simulink model "HarnessModel_ElevationProfile"  (R2026a)
settings: Solver=daessc  StopTime=40
PreLoadFcn:
  | setupHarness_ElevationProfile
values from neighbouring files (symbols this model uses):
  s = 100    [ElevationProfile_Description.m]
undefined symbols (not defined in the file or in its folder): initial, InputLUT, RoadSurface
libraries: fl_lib x12, nesl_utility x9, sdl_lib x4
settings Model: Creator=isaacito  LastModifiedBy=isaacito
settings SimscapeCC: SimscapeLogSimulationStatistics=on  SimscapeLogLimitData=off

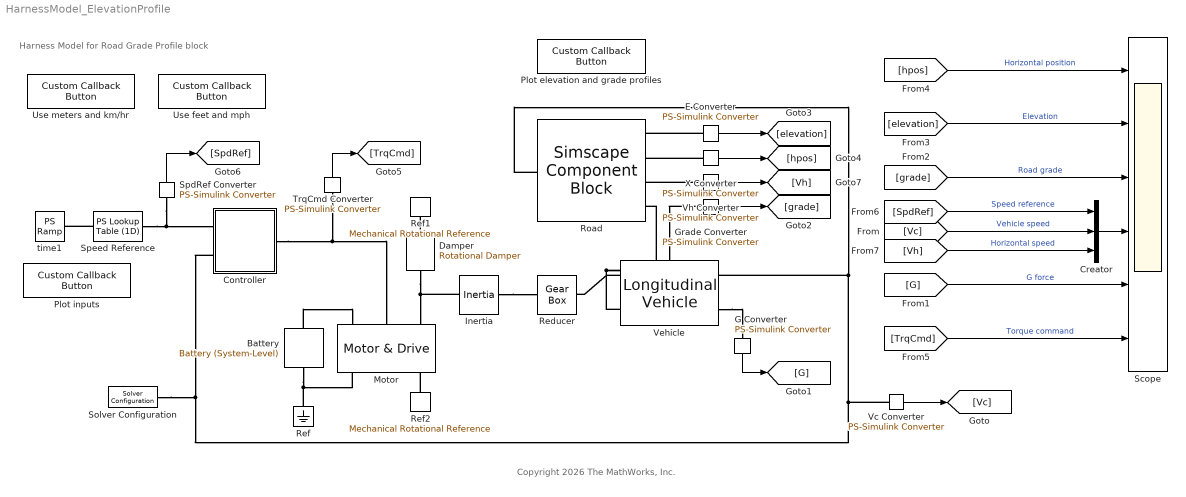
== system HarnessModel_ElevationProfile ==
  note: Harness Model for Road Grade Profile block
  note: Copyright 2026 The MathWorks, Inc.
  Battery : sdl_lib/Sources/Battery (System-Level)  Vnom=340 V  R1=0.01 Ohm  prm_AH=sdl.enum.InfiniteFinite.Infinite  AH=50 A*hr  V1=11.5 V  AH1=25 A*hr  prm_R2=sdl.enum.DisabledEnabled.Disabled  R2=2000 Ohm  thermal_port=simscape.enum.thermaleffects.omit  thermal_mass=30000 J/K  i_specify=off  i_priority=None  i=0 A  i_nominal_specify=off  i_nominal_value=1  i_nominal_unit=A  v_specify=off  v_priority=None  v=0 V  v_nominal_specify=off  v_nominal_value=1  v_nominal_unit=V  charge_specify=off  charge_priority=High  charge=50 A*hr  charge_nominal_specify=off  charge_nominal_value=1  charge_nominal_unit=A*hr  temperature_specify=off  temperature_priority=High  temperature=300 K  temperature_nominal_specify=off  temperature_nominal_value=1  temperature_nominal_unit=K
      settings: AttributesFormatString=%<Vnom> (%<Vnom_unit>)
  Controller : Subsystem
  Creator : BusCreator  Inputs=3
  Damper : sdl_lib/Couplings & Drives/Springs & Dampers/Rotational Damper  D=1e-5 N*m*s/rad  thermal_port=simscape.enum.thermaleffects.omit  thermal_mass=50 kJ/K  temperature_specify=off  temperature_priority=High  temperature=300 K  temperature_nominal_specify=off  temperature_nominal_value=1  temperature_nominal_unit=K
  E Converter : nesl_utility/PS-Simulink Converter  PhysicalDomain=network_engine_domain  SubClassName=ps_output  LeftPortType=input  RightPortType=output  PseudoPeriodic=off  Frequencies=[]  VectorFormat=inherit  Unit=ft  AffineConversion=off
  G Converter : nesl_utility/PS-Simulink Converter  PhysicalDomain=network_engine_domain  SubClassName=ps_output  LeftPortType=input  RightPortType=output  PseudoPeriodic=off  Frequencies=[]  VectorFormat=inherit  Unit=inherit  AffineConversion=off
  Grade Converter : nesl_utility/PS-Simulink Converter  PhysicalDomain=network_engine_domain  SubClassName=ps_output  LeftPortType=input  RightPortType=output  PseudoPeriodic=off  Frequencies=[]  VectorFormat=inherit  Unit=inherit  AffineConversion=off
  Inertia : fl_lib/Mechanical/Rotational Elements/Inertia  inertia=5*0.01^2 kg*m^2  num_ports=foundation.enum.numPorts2.two  w_specify=on  w_priority=None  w=0 rad/s  w_nominal_specify=off  w_nominal_value=1  w_nominal_unit=rad/s  t_specify=off  t_priority=None  t=0 N*m  t_nominal_specify=off  t_nominal_value=1  t_nominal_unit=N*m
      settings: AttributesFormatString=Priority: %<w_priority>
  Motor : sdl_lib/Engines & Motors/Motor & Drive  torque_max=160 N*m  power_max=90 kW  Tc=0.02 s  eff=100  w_eff=3750 rpm  T_eff=100 N*m  thermal_port=simscape.enum.thermaleffects.omit  thermal_mass=100 J/K  temperature_specify=off  temperature_priority=High  temperature=300 K  temperature_nominal_specify=off  temperature_nominal_value=1  temperature_nominal_unit=K
      settings: AttributesFormatString=|
      | %<torque_max> (%<torque_max_unit>)
      | %<power_max> (%<power_max_unit>)
  Plot elevation and grade profiles : CustomCallbackButton  Configuration="{\"components\":[{\"name\":\"BackgroundImageComponent\",\"settings\":{\"image\":{\"size\":[0,0],\"src\":\"default\",\"srcOrientation\":\"Right\"},\"position\":[0,0,1,1]}},{\"name\":\"ButtonStateComponent\",\"settings\":{\"buttonType\":\"momentary\",\"clickFcn\":\"plotRoadGradeProfileBlock( ...\\n  gcs + \\\"\\/Road\\\", ...\\n  UpdateModel = true, ... must update the model to get the latest values from the base workspace.\\n  InterpolationInterval = ...\\n    simscape.Value(0.2, \\\"m\\\"), ...\\n  PlotBaseData = true )\\n\",\"onValue\":1,\"position\":[0,0,1,1],\"pressDelay\":\"500\",\"pressFcn\":\"\",\"repeatInterval\":\"0\",\"states\":[{\"horizontalAlignment\":\"center\",\"image\":{\"position\":[0,0,1,1],\"size\":[1,1],\"src\":\"default\",\"srcOrientation\":\"Right\"},\"label\":{\"color\":[0.01176470588,0.01176470588,0.01176470588,1],\"icon\":{\"size\":[0,0],\"src\":\"default\",\"srcOrientation\":\"Right\"},\"iconOffset\":0,\"iconPlacement\":\"left\",\"opacity\":1,\"show\":true,\"text\":{\"content\":\"Plot profiles\",\"font\":\"Helvetica\"}},\"labelOffset\":[0,0],\"verticalAlignment\":\"middle\"},{\"horizontalAlignment\":\"center\",\"image\":{\"position\":[0,0,1,1],\"size\":[1,1],\"src\":\"default\",\"srcOrientation\":\"Right\"},\"label\":{\"color\":[0.01176470588,0.01176470588,0.01176470588,1],\"icon\":{\"size\":[0,0],\"src\":\"default\",\"srcOrientation\":\"Right\"},\"iconOffset\":0,\"iconPlacement\":\"left\",\"opacity\":1,\"show\":true,\"text\":{\"content\":\"Plot profiles\",\"font\":\"Helvetica\"}},\"labelOffset\":[0,0],\"verticalAlignment\":\"middle\"},{\"horizontalAlignment\":\"center\",\"image\":{\"position\":[0,0,1,1],\"size\":[1,1],\"src\":\"default\",\"srcOrientation\":\"Right\"},\"label\":{\"color\":[0.01176470588,0.01176470588,0.01176470588,1],\"icon\":{\"size\":[0,0],\"src\":\"default\",\"srcOrientation\":\"Right\"},\"iconOffset\":0,\"iconPlacement\":\"left\",\"opacity\":1,\"show\":true,\"text\":{\"content\":\"Plot profiles\",\"font\":\"Helvetica\"}},\"labelOffset\":[0,0],\"verticalAlignment\":\"middle\"},{\"horizontalAlignment\":\"center\",\"image\":{\"position\":[0,0,1,1],\"size\":[1,1],\"src\":\"default\",\"srcOrientation\":\"Right\"},\"label\":{\"color\":[0.01176470588,0.01176470588,0.01176470588,1],\"icon\":{\"size\":[0,0],\"src\":\"default\",\"srcOrientation\":\"Right\"},\"iconOffset\":0,\"iconPlacement\":\"left\",\"opacity\":1,\"show\":true,\"text\":{\"content\":\"Plot profiles\",\"font\":\"Helvetica\"}},\"labelOffset\":[0,0],\"verticalAlignment\":\"middle\"}]}},{\"name\":\"ForegroundImageComponent\",\"settings\":{\"image\":{\"size\":[0,0],\"src\":\"default\",\"srcOrientation\":\"Right\"},\"isForeground\":1,\"position\":[0,0,1,1]}}],\"derived\":{\"blockParameters\":{\"AutoActivate\":true,\"ButtonText\":\"Plot profiles\",\"ButtonType\":\"Momentary\",\"ClickFcn\":\"plotRoadGradeProfileBlock( ...\\n  gcs + \\\"\\/Road\\\", ...\\n  UpdateModel = true, ... must update the model to get the latest values from the base workspace.\\n  InterpolationInterval = ...\\n    simscape.Value(0.2, \\\"m\\\"), ...\\n  PlotBaseData = true )\\n\",\"OnValue\":1,\"PressDelay\":\"500\",\"PressFcn\":\"\",\"RepeatInterval\":\"0\",\"fixedAspectRatio\":\"off\"}},\"settings\":{\"BindingType\":\"standalone\",\"autoActivate\":true,\"backgroundColor\":[244,244,244,1],\"backgroundOffset\":0.2,\"backgroundOpacity\":1,\"fixedAspectRatio\":\"off\",\"foregroundColor\":[0.01176470588,0.01176470588,0.01176470588,1],\"migratedFromLegacy\":true,\"useBackgroundColor\":true,\"variant\":\"callback\",\"version\":\"R2025a\"},\"type\":\"Button\"}"  CustomBackgroundColor="{\"color\":[0.9568627451,0.9568627451,0.9568627451],\"show\":true}"
  Plot inputs : CustomCallbackButton  Configuration="{\"components\":[{\"name\":\"BackgroundImageComponent\",\"settings\":{\"image\":{\"size\":[0,0],\"src\":\"default\",\"srcOrientation\":\"Right\"},\"position\":[0,0,1,1]}},{\"name\":\"ButtonStateComponent\",\"settings\":{\"buttonType\":\"momentary\",\"clickFcn\":\"bevutil1.SignalUtil.plotLookupTable1DBlocks(...\\n  gcs, ...\\n  Blocks = \\\"Speed Reference\\\", ...\\n  UpdateModel = true, ... must update the model to get the latest values from the base workspace.\\n  DivisionType = \\\"InterpolationInterval\\\", ...\\n  InterpolationInterval = 0.05 )\\n\",\"onValue\":1,\"position\":[0,0,1,1],\"pressDelay\":\"500\",\"pressFcn\":\"\",\"repeatInterval\":\"0\",\"states\":[{\"horizontalAlignment\":\"center\",\"image\":{\"position\":[0,0,1,1],\"size\":[1,1],\"src\":\"default\",\"srcOrientation\":\"Right\"},\"label\":{\"color\":[0.01176470588,0.01176470588,0.01176470588,1],\"icon\":{\"size\":[0,0],\"src\":\"default\",\"srcOrientation\":\"Right\"},\"iconOffset\":0,\"iconPlacement\":\"left\",\"opacity\":1,\"show\":true,\"text\":{\"content\":\"Plot inputs\",\"font\":\"Helvetica\"}},\"labelOffset\":[0,0],\"verticalAlignment\":\"middle\"},{\"horizontalAlignment\":\"center\",\"image\":{\"position\":[0,0,1,1],\"size\":[1,1],\"src\":\"default\",\"srcOrientation\":\"Right\"},\"label\":{\"color\":[0.01176470588,0.01176470588,0.01176470588,1],\"icon\":{\"size\":[0,0],\"src\":\"default\",\"srcOrientation\":\"Right\"},\"iconOffset\":0,\"iconPlacement\":\"left\",\"opacity\":1,\"show\":true,\"text\":{\"content\":\"Plot inputs\",\"font\":\"Helvetica\"}},\"labelOffset\":[0,0],\"verticalAlignment\":\"middle\"},{\"horizontalAlignment\":\"center\",\"image\":{\"position\":[0,0,1,1],\"size\":[1,1],\"src\":\"default\",\"srcOrientation\":\"Right\"},\"label\":{\"color\":[0.01176470588,0.01176470588,0.01176470588,1],\"icon\":{\"size\":[0,0],\"src\":\"default\",\"srcOrientation\":\"Right\"},\"iconOffset\":0,\"iconPlacement\":\"left\",\"opacity\":1,\"show\":true,\"text\":{\"content\":\"Plot inputs\",\"font\":\"Helvetica\"}},\"labelOffset\":[0,0],\"verticalAlignment\":\"middle\"},{\"horizontalAlignment\":\"center\",\"image\":{\"position\":[0,0,1,1],\"size\":[1,1],\"src\":\"default\",\"srcOrientation\":\"Right\"},\"label\":{\"color\":[0.01176470588,0.01176470588,0.01176470588,1],\"icon\":{\"size\":[0,0],\"src\":\"default\",\"srcOrientation\":\"Right\"},\"iconOffset\":0,\"iconPlacement\":\"left\",\"opacity\":1,\"show\":true,\"text\":{\"content\":\"Plot inputs\",\"font\":\"Helvetica\"}},\"labelOffset\":[0,0],\"verticalAlignment\":\"middle\"}]}},{\"name\":\"ForegroundImageComponent\",\"settings\":{\"image\":{\"size\":[0,0],\"src\":\"default\",\"srcOrientation\":\"Right\"},\"isForeground\":1,\"position\":[0,0,1,1]}}],\"derived\":{\"blockParameters\":{\"AutoActivate\":true,\"ButtonText\":\"Plot inputs\",\"ButtonType\":\"Momentary\",\"ClickFcn\":\"bevutil1.SignalUtil.plotLookupTable1DBlocks(...\\n  gcs, ...\\n  Blocks = \\\"Speed Reference\\\", ...\\n  UpdateModel = true, ... must update the model to get the latest values from the base workspace.\\n  DivisionType = \\\"InterpolationInterval\\\", ...\\n  InterpolationInterval = 0.05 )\\n\",\"OnValue\":1,\"PressDelay\":\"500\",\"PressFcn\":\"\",\"RepeatInterval\":\"0\",\"fixedAspectRatio\":\"off\"}},\"settings\":{\"BindingType\":\"standalone\",\"autoActivate\":true,\"backgroundColor\":[244,244,244,1],\"backgroundOffset\":0.2,\"backgroundOpacity\":1,\"fixedAspectRatio\":\"off\",\"foregroundColor\":[0.01176470588,0.01176470588,0.01176470588,1],\"migratedFromLegacy\":true,\"useBackgroundColor\":true,\"variant\":\"callback\",\"version\":\"R2025a\"},\"type\":\"Button\"}"  CustomBackgroundColor="{\"color\":[0.9568627451,0.9568627451,0.9568627451],\"show\":true}"
  Reducer : fl_lib/Mechanical/Mechanisms/Gear Box  ratio=9.1  t_in_specify=off  t_in_priority=None  t_in=0 N*m  t_in_nominal_specify=off  t_in_nominal_value=1  t_in_nominal_unit=N*m  t_out_specify=off  t_out_priority=None  t_out=0 N*m  t_out_nominal_specify=off  t_out_nominal_value=1  t_out_nominal_unit=N*m
      settings: AttributesFormatString=%<ratio>
  Ref : fl_lib/Electrical/Electrical Elements/Electrical Reference
  Ref1 : fl_lib/Mechanical/Rotational Elements/Mechanical Rotational Reference
  Ref2 : fl_lib/Mechanical/Rotational Elements/Mechanical Rotational Reference
  Road : SimscapeComponentBlock  SourceFile=RoadGradeProfile  ComponentPath=RoadGradeProfile  ComponentVariants="[\"RoadGradeProfile\"]"  ComponentVariantNames="[\"RoadGradeProfile\"]"  ClassName=RoadGradeProfile  SchemaVersion=1  x_vector="RoadSurface.HorizontalDistance.value(\"m\") m"  grade_vector=RoadSurface.GradePercent  profile_interp_method=simscape.enum.interpolation.smooth  left_elevation="RoadSurface.LeftElevation.value(\"m\") m"  initial_position="initial.HorizontalPosition.value(\"m\") m"
      settings: CopyFcn=simscape.sscblock.internal.componentBlockCallback(gcbh,'COPY')  PreCopyFcn=simscape.sscblock.internal.componentBlockCallback(gcbh,'PRECOPY')  PreDeleteFcn=simscape.sscblock.internal.componentBlockCallback(gcbh,'PREDELETE')
      mask Type: Road Grade Profile
  Scope : Scope  NumInputPorts=6
      settings: ActiveDisplayString=4  ActiveDisplayYMinimum=-2.3333753364262253  ActiveDisplayYMaximum=21.000378027836032
  Solver Configuration : nesl_utility/Solver Configuration  PhysicalDomain=network_engine_domain  SubClassName=solver  LeftPortType=input  RightPortType=generic  Tones=[]  Harmonics=[]  SimulateNoise=off  Profile=off  UseLocalSampling=off  EnableSwitchedLinearOptims=on  FrequencyDomain=off  UseCCode=off  RelTol=0.001  AbsTol=0.001  MinStep=1e-09  ToWorkspace=off  RevertToSquareIcSolve=off  NumHomotopyIterations=100  PhasorMode=off  PhasorModeNumHarmonics=1  ConsistencySolver=NEWTON_XTOL_AFTER_FTOL  CanonicalOrdering=CANONICAL  OptimizeIntermediates=OPTIMIZED  IndexReductionMethod=DerivativeReplacement  DoDC=off  ResidualTolerance=1e-09  ConsistencyTolSource=GLOBAL  ConsistencyAbsTol=0.001  ConsistencyRelTol=0.001  ConsistencyTolFactor=0.001  UseLocalSolver=off  LocalSolverChoice=NE_BACKWARD_EULER_ADVANCER  ResolveIndetEquations=on  FunctionEvalNumThread=1  LocalSolverSampleTime=0.001  DoFixedCost=off  MaxNonlinIter=3  MaxModeIter=2  ComputeImpulses=off  ImpulseIterations=2  LinearAlgebra=auto  LinearAlgebraNumThread=0  EquationFormulation=NE_TIME_EF  DelaysMemoryBudget=1024  AutomaticFiltering=on  FilteringTimeConstant=0.001  PartitionStorageMethod=AS_NEEDED  PartitionMemoryBudget=1024  PartitionMethod=ROBUST  MultibodyUseLocalSolver=off  MultibodyLocalSolverChoice=ODE1  MultibodyLocalSolverSampleTime=0.001
      settings: AttributesFormatString=Local solver: %<UseLocalSolver>
  SpdRef Converter : nesl_utility/PS-Simulink Converter  PhysicalDomain=network_engine_domain  SubClassName=ps_output  LeftPortType=input  RightPortType=output  PseudoPeriodic=off  Frequencies=[]  VectorFormat=inherit  Unit=mph  AffineConversion=off
  Speed Reference : fl_lib/Physical Signals/Lookup Tables/PS Lookup Table (1D)  x="InputLUT.SpeedReference.Time.value(\"s\") s"  f="InputLUT.SpeedReference.Speed.value(\"km/hr\") km/hr"  interp_method=simscape.enum.interpolation.smooth  extrap_method=simscape.enum.extrapolation.nearest
  TrqCmd Converter : nesl_utility/PS-Simulink Converter  PhysicalDomain=network_engine_domain  SubClassName=ps_output  LeftPortType=input  RightPortType=output  PseudoPeriodic=off  Frequencies=[]  VectorFormat=inherit  Unit=inherit  AffineConversion=off
  Use feet and mph : CustomCallbackButton  Configuration="{\"components\":[{\"name\":\"BackgroundImageComponent\",\"settings\":{\"image\":{\"size\":[0,0],\"src\":\"default\",\"srcOrientation\":\"Right\"},\"position\":[0,0,1,1]}},{\"name\":\"ButtonStateComponent\",\"settings\":{\"buttonType\":\"momentary\",\"clickFcn\":\"set_param(gcs+\\\"\\/SpdRef Converter\\\", Unit=\\\"mph\\\")\\nset_param(gcs+\\\"\\/Vh Converter\\\", Unit=\\\"mph\\\")\\nset_param(gcs+\\\"\\/Vc Converter\\\", Unit=\\\"mph\\\")\\nset_param(gcs+\\\"\\/E Converter\\\", Unit=\\\"ft\\\")\\nset_param(gcs+\\\"\\/X Converter\\\", Unit=\\\"ft\\\")\\n\",\"onValue\":1,\"position\":[0,0,1,1],\"pressDelay\":\"500\",\"pressFcn\":\"\",\"repeatInterval\":\"0\",\"states\":[{\"horizontalAlignment\":\"center\",\"image\":{\"position\":[0,0,1,1],\"size\":[1,1],\"src\":\"default\",\"srcOrientation\":\"Right\"},\"label\":{\"color\":[0.01176470588,0.01176470588,0.01176470588,1],\"icon\":{\"size\":[0,0],\"src\":\"default\",\"srcOrientation\":\"Right\"},\"iconOffset\":0,\"iconPlacement\":\"left\",\"opacity\":1,\"show\":true,\"text\":{\"content\":\"Set units\",\"font\":\"Helvetica\"}},\"labelOffset\":[0,0],\"verticalAlignment\":\"middle\"},{\"horizontalAlignment\":\"center\",\"image\":{\"position\":[0,0,1,1],\"size\":[1,1],\"src\":\"default\",\"srcOrientation\":\"Right\"},\"label\":{\"color\":[0.01176470588,0.01176470588,0.01176470588,1],\"icon\":{\"size\":[0,0],\"src\":\"default\",\"srcOrientation\":\"Right\"},\"iconOffset\":0,\"iconPlacement\":\"left\",\"opacity\":1,\"show\":true,\"text\":{\"content\":\"Set units\",\"font\":\"Helvetica\"}},\"labelOffset\":[0,0],\"verticalAlignment\":\"middle\"},{\"horizontalAlignment\":\"center\",\"image\":{\"position\":[0,0,1,1],\"size\":[1,1],\"src\":\"default\",\"srcOrientation\":\"Right\"},\"label\":{\"color\":[0.01176470588,0.01176470588,0.01176470588,1],\"icon\":{\"size\":[0,0],\"src\":\"default\",\"srcOrientation\":\"Right\"},\"iconOffset\":0,\"iconPlacement\":\"left\",\"opacity\":1,\"show\":true,\"text\":{\"content\":\"Set units\",\"font\":\"Helvetica\"}},\"labelOffset\":[0,0],\"verticalAlignment\":\"middle\"},{\"horizontalAlignment\":\"center\",\"image\":{\"position\":[0,0,1,1],\"size\":[1,1],\"src\":\"default\",\"srcOrientation\":\"Right\"},\"label\":{\"color\":[0.01176470588,0.01176470588,0.01176470588,1],\"icon\":{\"size\":[0,0],\"src\":\"default\",\"srcOrientation\":\"Right\"},\"iconOffset\":0,\"iconPlacement\":\"left\",\"opacity\":1,\"show\":true,\"text\":{\"content\":\"Set units\",\"font\":\"Helvetica\"}},\"labelOffset\":[0,0],\"verticalAlignment\":\"middle\"}]}},{\"name\":\"ForegroundImageComponent\",\"settings\":{\"image\":{\"size\":[0,0],\"src\":\"default\",\"srcOrientation\":\"Right\"},\"isForeground\":1,\"position\":[0,0,1,1]}}],\"derived\":{\"blockParameters\":{\"AutoActivate\":true,\"ButtonText\":\"Set units\",\"ButtonType\":\"Momentary\",\"ClickFcn\":\"set_param(gcs+\\\"\\/SpdRef Converter\\\", Unit=\\\"mph\\\")\\nset_param(gcs+\\\"\\/Vh Converter\\\", Unit=\\\"mph\\\")\\nset_param(gcs+\\\"\\/Vc Converter\\\", Unit=\\\"mph\\\")\\nset_param(gcs+\\\"\\/E Converter\\\", Unit=\\\"ft\\\")\\nset_param(gcs+\\\"\\/X Converter\\\", Unit=\\\"ft\\\")\\n\",\"OnValue\":1,\"PressDelay\":\"500\",\"PressFcn\":\"\",\"RepeatInterval\":\"0\",\"fixedAspectRatio\":\"off\"}},\"settings\":{\"BindingType\":\"standalone\",\"autoActivate\":true,\"backgroundColor\":[244,244,244,1],\"backgroundOffset\":0.2,\"backgroundOpacity\":1,\"fixedAspectRatio\":\"off\",\"foregroundColor\":[0.01176470588,0.01176470588,0.01176470588,1],\"migratedFromLegacy\":true,\"useBackgroundColor\":true,\"variant\":\"callback\",\"version\":\"R2025a\"},\"type\":\"Button\"}"  CustomBackgroundColor="{\"color\":[0.9568627451,0.9568627451,0.9568627451],\"show\":true}"
  Use meters and km/hr : CustomCallbackButton  Configuration="{\"components\":[{\"name\":\"BackgroundImageComponent\",\"settings\":{\"image\":{\"size\":[0,0],\"src\":\"default\",\"srcOrientation\":\"Right\"},\"position\":[0,0,1,1]}},{\"name\":\"ButtonStateComponent\",\"settings\":{\"buttonType\":\"momentary\",\"clickFcn\":\"set_param(gcs+\\\"\\/SpdRef Converter\\\", Unit=\\\"km\\/hr\\\")\\nset_param(gcs+\\\"\\/Vh Converter\\\", Unit=\\\"km\\/hr\\\")\\nset_param(gcs+\\\"\\/Vc Converter\\\", Unit=\\\"km\\/hr\\\")\\nset_param(gcs+\\\"\\/E Converter\\\", Unit=\\\"m\\\")\\nset_param(gcs+\\\"\\/X Converter\\\", Unit=\\\"m\\\")\\n\",\"onValue\":1,\"position\":[0,0,1,1],\"pressDelay\":\"500\",\"pressFcn\":\"\",\"repeatInterval\":\"0\",\"states\":[{\"horizontalAlignment\":\"center\",\"image\":{\"position\":[0,0,1,1],\"size\":[1,1],\"src\":\"default\",\"srcOrientation\":\"Right\"},\"label\":{\"color\":[0.01176470588,0.01176470588,0.01176470588,1],\"icon\":{\"size\":[0,0],\"src\":\"default\",\"srcOrientation\":\"Right\"},\"iconOffset\":0,\"iconPlacement\":\"left\",\"opacity\":1,\"show\":true,\"text\":{\"content\":\"Set units\",\"font\":\"Helvetica\"}},\"labelOffset\":[0,0],\"verticalAlignment\":\"middle\"},{\"horizontalAlignment\":\"center\",\"image\":{\"position\":[0,0,1,1],\"size\":[1,1],\"src\":\"default\",\"srcOrientation\":\"Right\"},\"label\":{\"color\":[0.01176470588,0.01176470588,0.01176470588,1],\"icon\":{\"size\":[0,0],\"src\":\"default\",\"srcOrientation\":\"Right\"},\"iconOffset\":0,\"iconPlacement\":\"left\",\"opacity\":1,\"show\":true,\"text\":{\"content\":\"Set units\",\"font\":\"Helvetica\"}},\"labelOffset\":[0,0],\"verticalAlignment\":\"middle\"},{\"horizontalAlignment\":\"center\",\"image\":{\"position\":[0,0,1,1],\"size\":[1,1],\"src\":\"default\",\"srcOrientation\":\"Right\"},\"label\":{\"color\":[0.01176470588,0.01176470588,0.01176470588,1],\"icon\":{\"size\":[0,0],\"src\":\"default\",\"srcOrientation\":\"Right\"},\"iconOffset\":0,\"iconPlacement\":\"left\",\"opacity\":1,\"show\":true,\"text\":{\"content\":\"Set units\",\"font\":\"Helvetica\"}},\"labelOffset\":[0,0],\"verticalAlignment\":\"middle\"},{\"horizontalAlignment\":\"center\",\"image\":{\"position\":[0,0,1,1],\"size\":[1,1],\"src\":\"default\",\"srcOrientation\":\"Right\"},\"label\":{\"color\":[0.01176470588,0.01176470588,0.01176470588,1],\"icon\":{\"size\":[0,0],\"src\":\"default\",\"srcOrientation\":\"Right\"},\"iconOffset\":0,\"iconPlacement\":\"left\",\"opacity\":1,\"show\":true,\"text\":{\"content\":\"Set units\",\"font\":\"Helvetica\"}},\"labelOffset\":[0,0],\"verticalAlignment\":\"middle\"}]}},{\"name\":\"ForegroundImageComponent\",\"settings\":{\"image\":{\"size\":[0,0],\"src\":\"default\",\"srcOrientation\":\"Right\"},\"isForeground\":1,\"position\":[0,0,1,1]}}],\"derived\":{\"blockParameters\":{\"AutoActivate\":true,\"ButtonText\":\"Set units\",\"ButtonType\":\"Momentary\",\"ClickFcn\":\"set_param(gcs+\\\"\\/SpdRef Converter\\\", Unit=\\\"km\\/hr\\\")\\nset_param(gcs+\\\"\\/Vh Converter\\\", Unit=\\\"km\\/hr\\\")\\nset_param(gcs+\\\"\\/Vc Converter\\\", Unit=\\\"km\\/hr\\\")\\nset_param(gcs+\\\"\\/E Converter\\\", Unit=\\\"m\\\")\\nset_param(gcs+\\\"\\/X Converter\\\", Unit=\\\"m\\\")\\n\",\"OnValue\":1,\"PressDelay\":\"500\",\"PressFcn\":\"\",\"RepeatInterval\":\"0\",\"fixedAspectRatio\":\"off\"}},\"settings\":{\"BindingType\":\"standalone\",\"autoActivate\":true,\"backgroundColor\":[244,244,244,1],\"backgroundOffset\":0.2,\"backgroundOpacity\":1,\"fixedAspectRatio\":\"off\",\"foregroundColor\":[0.01176470588,0.01176470588,0.01176470588,1],\"migratedFromLegacy\":true,\"useBackgroundColor\":true,\"variant\":\"callback\",\"version\":\"R2025a\"},\"type\":\"Button\"}"  CustomBackgroundColor="{\"color\":[0.9568627451,0.9568627451,0.9568627451],\"show\":true}"
  Vc Converter : nesl_utility/PS-Simulink Converter  PhysicalDomain=network_engine_domain  SubClassName=ps_output  LeftPortType=input  RightPortType=output  PseudoPeriodic=off  Frequencies=[]  VectorFormat=inherit  Unit=mph  AffineConversion=off
  Vehicle : sdl_lib/Tires & Vehicles/Longitudinal Vehicle  vehParamType=sdl.enum.VehicleParameterizationType.Regular  M_vehicle=1800 kg  R_tireroll=0.34 m  C_tireroll=0.013  C_airdrag=0.34  A_front=2.5 m^2  A_rl=120 N  B_rl=1.8 N*s/m  C_rl=0.389 N*s^2/m^2  g=9.81 m/s^2  V_1=0.1 m/s  w_1=0.1 rad/s  ShowBrakeIn=false  ShowSlopeIn=true  SlopeInputType=sdl.enum.VehicleLongitudinalRoadSlopeInputType.GradePercent  ShowWindIn=false  ShowGOut=true  air_density=1.184 kg/m^3  V_x_specify=on  V_x_priority=High  V_x=0 km/hr  V_x_nominal_specify=off  V_x_nominal_value=1  V_x_nominal_unit=m/s  trq_specify=off  trq_priority=None  trq=0 N*m  trq_nominal_specify=off  trq_nominal_value=1  trq_nominal_unit=N*m  w_specify=off  w_priority=None  w=0 rad/s  w_nominal_specify=off  w_nominal_value=1  w_nominal_unit=rad/s
      settings: AttributesFormatString=Initial: %<V_x> (%<V_x_unit>)
  Vh Converter : nesl_utility/PS-Simulink Converter  PhysicalDomain=network_engine_domain  SubClassName=ps_output  LeftPortType=input  RightPortType=output  PseudoPeriodic=off  Frequencies=[]  VectorFormat=inherit  Unit=mph  AffineConversion=off
  X Converter : nesl_utility/PS-Simulink Converter  PhysicalDomain=network_engine_domain  SubClassName=ps_output  LeftPortType=input  RightPortType=output  PseudoPeriodic=off  Frequencies=[]  VectorFormat=inherit  Unit=ft  AffineConversion=off
  time1 : fl_lib/Physical Signals/Sources/PS Ramp  slope=1  start_time=0 s  initial_output=0 s  ZeroCross=false
  wires:
  [hpos] -> Scope/1  "Horizontal position"
  [elevation] -> Scope/2  "Elevation"
  [grade] -> Scope/3  "Road grade"
  [G] -> Scope/5  "G force"
  [TrqCmd] -> Scope/6  "Torque command"
  [SpdRef] -> Creator/1  "Speed reference"
  [Vc] -> Creator/2  "Vehicle speed"
  Creator/1 -> Scope/4
  Grade Converter/1 -> [grade]
  Vh Converter/1 -> [Vh]
  X Converter/1 -> [hpos]
  E Converter/1 -> [elevation]
  G Converter/1 -> [G]
  SpdRef Converter/1 -> [SpdRef]
  Vc Converter/1 -> [Vc]
  TrqCmd Converter/1 -> [TrqCmd]
  [Vh] -> Creator/3  "Horizontal speed"
  connections:
  Vehicle/LConn1 -- Reducer/RConn1
  Controller/LConn2 -- Road/LConn1 -- Vehicle/RConn1 -- Vc Converter/LConn1 -- Solver Configuration/RConn1
  Vehicle/LConn2 -- Road/RConn4 -- Grade Converter/LConn1
  Battery/LConn1 -- Motor/LConn1
  Battery/RConn1 -- Motor/RConn1 -- Ref/LConn1
  Inertia/LConn1 -- Reducer/LConn1
  Inertia/RConn1 -- Damper/LConn1 -- Motor/LConn3
  Ref2/LConn1 -- Motor/RConn3
  Damper/RConn1 -- Ref1/LConn1
  Controller/RConn1 -- TrqCmd Converter/LConn1 -- Motor/LConn2
  Speed Reference/LConn1 -- time1/RConn1
  Speed Reference/RConn1 -- Controller/LConn1 -- SpdRef Converter/LConn1
  Vh Converter/LConn1 -- Road/RConn3
  X Converter/LConn1 -- Road/RConn2
  E Converter/LConn1 -- Road/RConn1
  Vehicle/RConn2 -- G Converter/LConn1

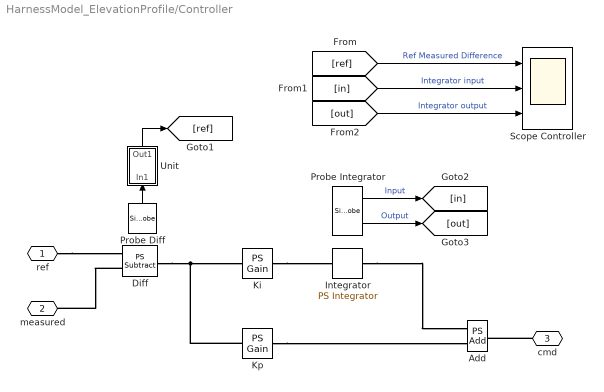
== system HarnessModel_ElevationProfile/Controller ==
  Add : fl_lib/Physical Signals/Functions/PS Add
  Diff : fl_lib/Physical Signals/Functions/PS Subtract
  Integrator : fl_lib/Physical Signals/Linear Operators/PS Integrator  reset_method=foundation.enum.IntegratorResetSpec.None  initial_condition_spec=foundation.enum.IntegratorICSpec.Internal  saturation_spec=foundation.enum.IntegratorSaturationSpec.None  saturation_source_spec=foundation.enum.IntegratorSaturationSourceSpec.Internal  x0=0 N*m  xu=1000 N*m  xl=-1000 N*m
      settings: AttributesFormatString=%<x0_unit>
  Ki : fl_lib/Physical Signals/Functions/PS Gain  gain=0 N
      settings: AttributesFormatString=%<gain_unit>
  Kp : fl_lib/Physical Signals/Functions/PS Gain  gain=2000 N*s
      settings: AttributesFormatString=%<gain_unit>
  Probe Diff : SimscapeProbe  BoundBlock=96  Variables="{\"O\":{\"Probing\":\"ON\"}}"
  Probe Integrator : SimscapeProbe  BoundBlock=90  Variables="{\"I\":{\"Probing\":\"ON\"},\"O\":{\"Probing\":\"ON\"}}"
  Scope Controller : Scope  NumInputPorts=3
      settings: ActiveDisplayYMinimum=-1  ActiveDisplayYMaximum=1
  Unit : Subsystem
  ref : PMIOPort  Side=Left
  measured : PMIOPort  Port=2  Side=Left
  cmd : PMIOPort  Port=3  Side=Right
  wires:
  Probe Diff/1 -> Unit/1(In1)
  Unit/1(Out1) -> [ref]
  Probe Integrator/1 -> [in]  "Input"
  Probe Integrator/2 -> [out]  "Output"
  [ref] -> Scope Controller/1  "Ref Measured Difference"
  [in] -> Scope Controller/2  "Integrator input"
  [out] -> Scope Controller/3  "Integrator output"
  connections:
  cmd/RConn1 -- Add/RConn1
  Integrator/RConn1 -- Add/LConn1
  Kp/RConn1 -- Add/LConn2
  Ki/RConn1 -- Integrator/LConn1
  Diff/RConn1 -- Kp/LConn1 -- Ki/LConn1
  Diff/LConn2 -- measured/RConn1
  ref/RConn1 -- Diff/LConn1

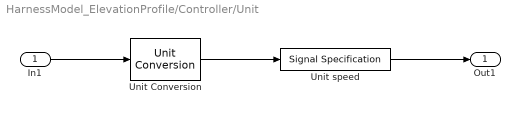
== system HarnessModel_ElevationProfile/Controller/Unit ==
  In1 : Inport
  Unit Conversion : UnitConversion
  Unit speed : SignalSpecification  Unit=km/hr
  Out1 : Outport
  wires:
  In1/1 -> Unit Conversion/1
  Unit speed/1 -> Out1/1
  Unit Conversion/1 -> Unit speed/1
